simulink model "outtest"  (Simulink 4.00)
settings: Solver=ode45  StartTime=0.0  StopTime=10.0  RelTol=1e-3
libraries: simulink3 x1
settings Model: Creator=mcar  LastModifiedBy=mcar  BlockReductionOpt=off

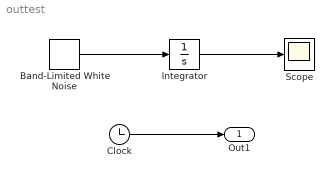
== system outtest ==
  Band-Limited White Noise : simulink3/Sources/Band-Limited White Noise  Cov=[0.1]  Ts=0.1  seed=[23341]
  Clock : Clock
      settings: DisplayTime=off  Decimation=10
  Integrator : Integrator  ExternalReset=none  InitialConditionSource=internal  InitialCondition=0  LimitOutput=off  UpperSaturationLimit=inf  LowerSaturationLimit=-inf  ShowSaturationPort=off  ShowStatePort=off  AbsoluteTolerance=auto
  Scope : Scope
      settings: TimeRange=auto  YMin=-5  YMax=5  SaveToWorkspace=off  SaveName=ScopeData  LimitDataPoints=on  MaxDataPoints=5000
  Out1 : Outport  Port=1
  wires:
  Integrator/1 -> Scope/1
  Band-Limited White Noise/1 -> Integrator/1
  Clock/1 -> Out1/1
